simulink model "ecu_deb"  (R2026a)
settings: Solver=FixedStepDiscrete  StopTime=10  FixedStep=0.001  SampleTimeConstraint=STIndependent
Description:
  | Fault debounce and healing. Source of truth for firmware/gen/ecu_deb.
settings Model: Creator=jj1001000  LastModifiedBy=jj1001000
settings OptimizationCC: DefaultUnderspecifiedDataType=single
settings DebuggingCC: ParameterPrecisionLossMsg=none
settings HardwareCC: ProdLargestAtomicInteger=Long  ProdLargestAtomicFloat=Double  ProdHWDeviceType=ARM Compatible->ARM Cortex-M
settings RTWCC: SystemTargetFile=ert.tlc  GenCodeOnly=on  Description=Embedded Coder
settings ERTTargetCC: UtilityFuncGeneration=Shared location  IncludeMdlTerminateFcn=off  CodeInterfacePackaging=Reusable function  SupportNonFinite=off

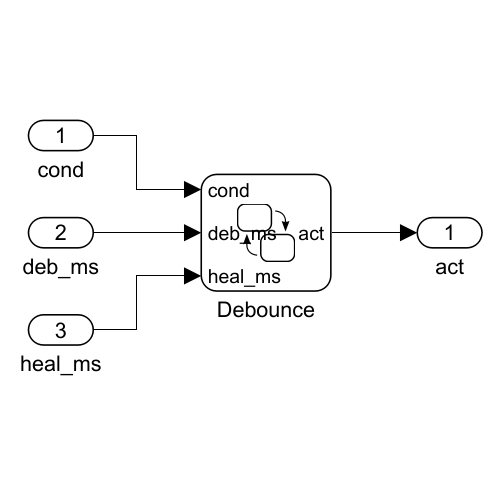
[thumbnail: Simulink's stored preview of the top-level diagram]
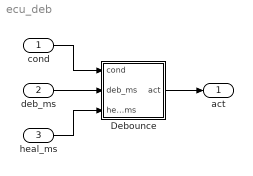
== system ecu_deb ==
  cond : Inport  OutDataTypeStr=uint8
  deb_ms : Inport  Port=2  OutDataTypeStr=uint16
  heal_ms : Inport  Port=3  OutDataTypeStr=uint16
  Debounce : Stateflow chart  TreatAsAtomicUnit=on
  act : Outport  OutDataTypeStr=uint8
  wires:
  cond/1 -> Debounce/1(cond)
  Debounce/1(act) -> act/1
  heal_ms/1 -> Debounce/3(heal_ms)
  deb_ms/1 -> Debounce/2(deb_ms)

== stateflow chart ecu_deb/Debounce ==
  settings: updateMethod=DISCRETE  executeAtInitialization=1
  state CLEAR
    entry: act = uint8(0);
    during: if cond ~= 0, n = n + uint16(1); else, n = uint16(0); end
  state ACTIVE
    entry: act = uint8(1);
    during: if cond == 0, n = n + uint16(1); else, n = uint16(0); end
  (default) -> CLEAR : {n = uint16(0); act = uint8(0);}
  CLEAR -> ACTIVE : [cond ~= 0 && n + uint16(1) >= deb_ms]{n = uint16(0);}
  ACTIVE -> CLEAR : [cond == 0 && n + uint16(1) >= heal_ms]{n = uint16(0);}
  data: cond input uint8; deb_ms input uint16; heal_ms input uint16; act output uint8; n local uint16
